simulink model "ffstudio_v2_6dof"  (R2026b)
settings: Solver=ode45  StopTime=25  MaxStep=0.02  RelTol=1e-6  AbsTol=1e-7
PostLoadFcn:
  | addpath(fileparts(fileparts(get_param('ffstudio_v2_6dof','FileName'))),'-begin');
model workspace (MAT data in the model file):
  ffStudioSimConfig.config.schemaVersion = 2
  ffStudioSimConfig.config.name = 'Blazhevski 6000 kg land-based firefighter'
  ffStudioSimConfig.config.designYear = 2036
  ffStudioSimConfig.config.payload_kg = 6000
  ffStudioSimConfig.config.crew_kg = 200
  ffStudioSimConfig.config.radius_km = 700
  ffStudioSimConfig.config.cruise_kmh = 580
  ffStudioSimConfig.config.cruiseAltitude_m = 5500
  ffStudioSimConfig.config.drop_kmh = 220
  ffStudioSimConfig.config.dropHeight_m = 40
  ffStudioSimConfig.config.pattern_min = 10
  ffStudioSimConfig.config.loiter_min = 45
  ffStudioSimConfig.config.loiter_kmh = 300
  ffStudioSimConfig.config.loiterAltitude_m = 1500
  ffStudioSimConfig.config.aspectRatio = 11.5
  ffStudioSimConfig.config.oswald = 0.8
  ffStudioSimConfig.config.wettedRatio = 5.5
  ffStudioSimConfig.config.KLD = 11
  ffStudioSimConfig.config.wingLoading_Nm2 = 3500
  ffStudioSimConfig.config.powerLoading_kWkg = 0.23
  ffStudioSimConfig.config.propEfficiency = 0.8
  ffStudioSimConfig.config.sfcCruise_kgkWh = 0.3
  ffStudioSimConfig.config.sfcLoiter_kgkWh = 0.36
  ffStudioSimConfig.config.takeoffFraction = 0.97
  ffStudioSimConfig.config.climbFraction = 0.985
  ffStudioSimConfig.config.descentFraction = 0.995
  ffStudioSimConfig.config.landingFraction = 0.995
  ffStudioSimConfig.config.reserveFactor = 1.06
  ffStudioSimConfig.config.emptyA = 1.442
  ffStudioSimConfig.config.emptyC = -0.0947
  ffStudioSimConfig.config.emptyScale = 1
  ffStudioSimConfig.config.sweepFactor = 1
  ffStudioSimConfig.config.gravity = 9.81
  ffStudioSimConfig.config.CLmaxClean = 1.6
  ffStudioSimConfig.config.CLmaxTakeoff = 2
  ffStudioSimConfig.config.CLmaxLanding = 2.4
  ffStudioSimConfig.config.deltaCDpattern = 0.06
  ffStudioSimConfig.config.deltaCDloiter = 0
  ffStudioSimConfig.config.powerLapseExponent = 0.7
  ffStudioSimConfig.config.engineCount = 2
  ffStudioSimConfig.config.takeoffTarget_m = 1000
  ffStudioSimConfig.config.landingTarget_m = 1000
  ffStudioSimConfig.config.climbTarget_ms = 8
  ffStudioSimConfig.config.oeiGradient = 0.024
  ffStudioSimConfig.config.muRoll = 0.03
  ffStudioSimConfig.config.muBrake = 0.35
  ffStudioSimConfig.config.deltaISA_K = 0
  ffStudioSimConfig.config.fieldAltitude_m = 0
  ffStudioSimConfig.config.taper = 0.45
  ffStudioSimConfig.config.tailArmH_m = 10.5
  ffStudioSimConfig.config.tailArmV_m = 10.2
  ffStudioSimConfig.config.VH = 1.106
  ffStudioSimConfig.config.VV = 0.0753
  ffStudioSimConfig.config.dihedral_deg = 2.75
  ffStudioSimConfig.config.aileronSpanFraction = 0.28
  ffStudioSimConfig.config.aileronChordFraction = 0.29
  ffStudioSimConfig.config.elevatorChordFraction = 0.34
  ffStudioSimConfig.config.rudderChordFraction = 0.335
  ffStudioSimConfig.config.cgEmpty_MAC = 0.28
  ffStudioSimConfig.config.cgCrew_MAC = -0.6
  ffStudioSimConfig.config.cgFuel_MAC = 0.3
  ffStudioSimConfig.config.cgWater_MAC = 0.3
  ffStudioSimConfig.config.cgMin_MAC = 0.15
  ffStudioSimConfig.config.cgMax_MAC = 0.4
  ffStudioSimConfig.config.dropDuration_s = 8
  ffStudioSimConfig.config.windNED_ms = [0 5 0]
  ffStudioSimConfig.config.parcelDiameter_m = 0.005
  ffStudioSimConfig.config.parcelCd = 0.47
  ffStudioSimConfig.config.waterDensity_kgm3 = 1000
  ffStudioSimConfig.config.releaseDown_ms = 0
  ffStudioSimConfig.config.releaseCount = 21
  ffStudioSimConfig.config.dyn.CL0 = 0.35
  ffStudioSimConfig.config.dyn.flapCL0 = 0.8
  ffStudioSimConfig.config.dyn.CLa = 5.2
  ffStudioSimConfig.config.dyn.CLde = 0.45
  ffStudioSimConfig.config.dyn.CLq = 3.5
  ffStudioSimConfig.config.dyn.Cm0 = 0
  ffStudioSimConfig.config.dyn.Cma = -0.8
  ffStudioSimConfig.config.dyn.Cmde = -1.1
  ffStudioSimConfig.config.dyn.Cmq = -12
  ffStudioSimConfig.config.dyn.CYb = -0.7
  ffStudioSimConfig.config.dyn.CYdr = 0.18
  ffStudioSimConfig.config.dyn.Clb = -0.1
  ffStudioSimConfig.config.dyn.Clp = -0.45
  ffStudioSimConfig.config.dyn.Clda = 0.18
  ffStudioSimConfig.config.dyn.Cnb = 0.15
  ffStudioSimConfig.config.dyn.Cnr = -0.2
  ffStudioSimConfig.config.dyn.Cndr = -0.12
  ffStudioSimConfig.config.dyn.radiusGyration_m = [5 6 7]
  ffStudioSimConfig.config.dyn.dropStart_s = 5
  ffStudioSimConfig.config.dyn.stopTime_s = 25
  ffStudioSimConfig.config.dyn.speedGain = 0.025
  ffStudioSimConfig.config.dyn.heightGain = 0.0015
  ffStudioSimConfig.config.dyn.pitchGain = 0.9
  ffStudioSimConfig.config.dyn.pitchRateGain = 0.5
  ffStudioSimConfig.config.dyn.rollGain = 0.6
  ffStudioSimConfig.config.dyn.rollRateGain = 0.3
  ffStudioSimConfig.config.dyn.yawRateGain = 0.4
  ffStudioSimConfig.config.dyn.fuelFlow_kgs = 0.2
  ffStudioSimConfig.config.dyn.autopilot = 1
  ffStudioSimConfig.config.dyn.engineOut = 0
  ffStudioSimConfig.config.dyn.elevatorPulse_deg = 0
  ffStudioSimConfig.config.dyn.pulseStart_s = 2
  ffStudioSimConfig.config.dyn.pulseDuration_s = 1
  ffStudioSimConfig.design.mtow_kg = 21965.2847244
  ffStudioSimConfig.design.fuel_kg = 3475.63176107
  ffStudioSimConfig.design.empty_kg = 12289.652954
  ffStudioSimConfig.design.payload_kg = 6000
  ffStudioSimConfig.design.crew_kg = 200
  ffStudioSimConfig.design.emptyFraction = 0.559503466867
  ffStudioSimConfig.design.payloadFraction = 0.273158307543
  ffStudioSimConfig.design.fuelFraction = 0.158232948249
  ffStudioSimConfig.design.wingArea_m2 = 61.5655551846
  ffStudioSimConfig.design.span_m = 26.6083423877
  ffStudioSimConfig.design.installedPower_kW = 5052.01548661
  ffStudioSimConfig.design.perEnginePower_kW = 2526.0077433
  ffStudioSimConfig.design.residual_kg = 9.29757698032e-06
  ffStudioSimConfig.design.mission.stations_kg = [21965.2847244; 21306.3261826; 20986.7312899; 20063.8378568; 19963.5186675; 19883.063741; 13883.063741; 13674.8177848; 13073.4664187; 13008.0990866; 12750.1375242; 12686.3868366]
  ffStudioSimConfig.design.mission.burn_kg = 3278.8978878
  ffStudioSimConfig.design.mission.fuel_kg = 3475.63176107
  ffStudioSimConfig.design.mission.extraReserve_kg = 196.733873268
  ffStudioSimConfig.design.mission.mode = 'report'
  ffStudioSimConfig.design.mission.table = table
  ffStudioSimConfig.design.mission.table.data{1} = [0; 1; 2; 3; 4; 5; 6; 7; 8; 9; 10]
  ffStudioSimConfig.design.mission.table.data{2} = [1; 2; 3; 4; 5; 6; 7; 8; 9; 10; 11]
  ffStudioSimConfig.design.mission.table.data{3} = ["Warm-up / taxi / take-off"; "Loaded climb"; "Outbound cruise"; "Descent to drop"; "Low-level pattern"; "Water release"; "Empty climb"; "Return cruise"; "Descent to reserve"; "Reserve loiter"; "Landing / taxi"]
  ffStudioSimConfig.design.mission.table.data{4} = [21965.2847244; 21306.3261826; 20986.7312899; 20063.8378568; 19963.5186675; 19883.063741; 13883.063741; 13674.8177848; 13073.4664187; 13008.0990866; 12750.1375242]
  ffStudioSimConfig.design.mission.table.data{5} = [21306.3261826; 20986.7312899; 20063.8378568; 19963.5186675; 19883.063741; 13883.063741; 13674.8177848; 13073.4664187; 13008.0990866; 12750.1375242; 12686.3868366]
  ffStudioSimConfig.design.mission.table.data{6} = [0.97; 0.985; 0.956024908294; 0.995; 0.995969902505; NaN; 0.985; 0.956024908294; 0.995; 0.980169157638; 0.995]
  ffStudioSimConfig.design.mission.table.data{7} = [658.958541731; 319.59489274; 922.89343308; 100.319189284; 80.4549265723; 0; 208.245956114; 601.35136615; 65.3673320935; 257.961562416; 63.7506876209]
  ffStudioSimConfig.design.mission.table.data{8} = [NaN; NaN; 4344.82758621; NaN; 600; 0; NaN; 4344.82758621; NaN; 2700; NaN]
  ffStudioSimConfig.design.mission.table.data{9} = [NaN; NaN; 3733.92048983; NaN; 1671.62217164; NaN; NaN; 3428.80965957; NaN; 932.367301197; NaN]
  ffStudioSimConfig.design.mission.table.data{10} = [NaN; NaN; 3404.69572299; NaN; 5038.44738929; NaN; NaN; 3404.69572299; NaN; 4559.620527; NaN]
  ffStudioSimConfig.design.mission.table.data{11} = [NaN; NaN; 15.9059737206; NaN; 11.1341816044; NaN; NaN; 15.9059737206; NaN; 13.774573242; NaN]
  ffStudioSimConfig.design.mission.table.data{12} = [NaN; NaN; 0.369620967159; NaN; 1.39601581167; NaN; NaN; 0.240842621252; NaN; 0.564188541196; NaN]
  ffStudioSimConfig.design.mission.table.ndims = 2
  ffStudioSimConfig.design.mission.table.nrows = 11
  ffStudioSimConfig.design.mission.table.nvars = 12
  ffStudioSimConfig.design.mission.table.varnames = {'From', 'To', 'Phase', 'Start_kg', 'End_kg', 'MassFraction', 'FuelBurn_kg', 'Duration_s', 'RequiredPower_kW', 'AvailablePower_kW', 'LD', 'CL'}
  ffStudioSimConfig.design.mission.table.props.CustomProps = struct()
  ffStudioSimConfig.design.mission.table.props.VariableCustomProps = struct()
  ffStudioSimConfig.design.mission.table.props.versionSavedFrom = 5
  ffStudioSimConfig.design.mission.table.props.minCompatibleVersion = 1
  ffStudioSimConfig.design.mission.table.props.incompatibilityMsg = ''
  ffStudioSimConfig.design.mission.table.props.VersionSavedFrom = 5
  ffStudioSimConfig.design.mission.table.props.useVariableNamesOriginal = 0
  ffStudioSimConfig.design.mission.table.props.useVariableNames2048 = 0
  ffStudioSimConfig.design.mission.table.props.useDimensionNamesOriginal = 0
  ffStudioSimConfig.design.mission.table.props.useDimensionNames2048 = 0
  ffStudioSimConfig.design.mission.table.props.Description = ''
  ffStudioSimConfig.design.mission.table.props.VariableNamesOriginal = {}
  ffStudioSimConfig.design.mission.table.props.VariableNames2048 = {}
  ffStudioSimConfig.design.mission.table.props.DimensionNames = {'Row', 'Variables'}
  ffStudioSimConfig.design.mission.table.props.DimensionNamesOriginal = {}
  ffStudioSimConfig.design.mission.table.props.DimensionNames2048 = {}
  ffStudioSimConfig.design.mission.table.props.UserData = []
  ffStudioSimConfig.design.mission.table.props.VariableDescriptions = {}
  ffStudioSimConfig.design.mission.table.props.VariableUnits = {}
  ffStudioSimConfig.design.mission.table.props.VariableContinuity = {}
  ffStudioSimConfig.design.mission.note = 'Climb/ground/descent/landing retain empirical report fractions. Requested speeds are checked against power availability, not automatically reduced.'
  ffStudioSimConfig.design.mode = 'report'
  ffStudioSimConfig.design.iteration = table
  ffStudioSimConfig.design.iteration.data = {[7200; 10128.8135593; 13057.6271186; 15986.440678; 18915.2542373; 21844.0677966; 24772.8813559; 27701.6949153; 30630.5084746; 33559.3220339; 36488.1355932; 39416.9491525; 42345.7627119; 45274.5762712; 48203.3898305; 51132.2033898; 54061.0169492; 56989.8305085; 59918.6440678; 62847.4576271; 65776.2711864; 68705.0847458; 71633.8983051; 74562.7118644; 77491.5254237; 80420.3389831; 83349.1525424; 86277.9661017; 89206.779661; 92135.5932203; 95064.4067797; 97993.220339; 100922.033898; 103850.847458; 106779.661017; 109708.474576; 112637.288136; 115566.101695; 118494.915254; 121423.728814; 124352.542373; 127281.355932; 130210.169492; 133138.983051; 136067.79661; 138996.610169; 141925.423729; 144854.237288; 147783.050847; 150711.864407; 153640.677966; 156569.491525; 159498.305085; 162427.118644; 165355.932203; 168284.745763; 171213.559322; 174142.372881; 177071.186441; 180000], [-4247.98280058; -3476.62310134; -2660.82656192; -1811.60280364; -935.682153221; -37.5963688103; 879.400809852; 1812.86331818; 2760.88747666; 3721.95108369; 4694.81021348; 5678.43002022; 6671.93663348; 7674.58269474; 8685.72203078; 9704.79063173; 10731.2920919; 11764.7862807; 12804.8803977; 13851.2218175; 14903.4922995; 15961.4032536; 17024.691831; 18093.1176703; 19166.4601655; 20244.5161577; 21327.09797; 22414.0317252; 23505.1558976; 24600.3200588; 25699.383787; 26802.2157136; 27908.6926868; 29018.6990337; 30132.1259087; 31248.870714; 32368.8365841; 33491.9319245; 34618.0699992; 35747.1685587; 36879.1495058; 38013.9385932; 39151.4651492; 40291.6618292; 41434.4643893; 42579.8114801; 43727.6444577; 44877.9072114; 46030.5460052; 47185.509332; 48342.7477802; 49502.2139094; 50663.8621371; 51827.6486328; 52993.5312202; 54161.469287; 55331.4237003; 56503.3567285; 57677.2319685; 58853.0142775]}
  ffStudioSimConfig.design.iteration.ndims = 2
  ffStudioSimConfig.design.iteration.nrows = 60
  ffStudioSimConfig.design.iteration.nvars = 2
  ffStudioSimConfig.design.iteration.varnames = {'AssumedMTOW_kg', 'ClosureResidual_kg'}
  ffStudioSimConfig.design.iteration.props.CustomProps = struct()
  ffStudioSimConfig.design.iteration.props.VariableCustomProps = struct()
  ffStudioSimConfig.design.iteration.props.versionSavedFrom = 5
  ffStudioSimConfig.design.iteration.props.minCompatibleVersion = 1
  ffStudioSimConfig.design.iteration.props.incompatibilityMsg = ''
  ffStudioSimConfig.design.iteration.props.VersionSavedFrom = 5
  ffStudioSimConfig.design.iteration.props.useVariableNamesOriginal = 0
  ffStudioSimConfig.design.iteration.props.useVariableNames2048 = 0
  ffStudioSimConfig.design.iteration.props.useDimensionNamesOriginal = 0
  ffStudioSimConfig.design.iteration.props.useDimensionNames2048 = 0
  ffStudioSimConfig.design.iteration.props.Description = ''
  ffStudioSimConfig.design.iteration.props.VariableNamesOriginal = {}
  ffStudioSimConfig.design.iteration.props.VariableNames2048 = {}
  ffStudioSimConfig.design.iteration.props.DimensionNames = {'Row', 'Variables'}
  ffStudioSimConfig.design.iteration.props.DimensionNamesOriginal = {}
  ffStudioSimConfig.design.iteration.props.DimensionNames2048 = {}
  ffStudioSimConfig.design.iteration.props.UserData = []
  ffStudioSimConfig.design.iteration.props.VariableDescriptions = {}
  ffStudioSimConfig.design.iteration.props.VariableUnits = {}
  ffStudioSimConfig.design.iteration.props.VariableContinuity = {}
  ffStudioSimConfig.polar.LDmax = 15.9059737206
  ffStudioSimConfig.polar.k = 0.0345989006722
  ffStudioSimConfig.polar.CD0 = 0.0285599332145
  ffStudioSimConfig.polar.CLbest = 0.908547094342
  ffStudioSimConfig.polar.CL = [0; 0.01; 0.02; 0.03; 0.04; 0.05; 0.06; 0.07; 0.08; 0.09; 0.1; 0.11; 0.12; 0.13; 0.14; 0.15; 0.16; 0.17; 0.18; 0.19; 0.2; 0.21; 0.22; 0.23; 0.24; 0.25; 0.26; 0.27; 0.28; 0.29; 0.3; 0.31; 0.32; 0.33; 0.34; 0.35; 0.36; 0.37; 0.38; 0.39; 0.4; 0.41; 0.42; 0.43; 0.44; 0.45; 0.46; 0.47; 0.48; 0.49; 0.5; 0.51; 0.52; 0.53; 0.54; 0.55; 0.56; 0.57; 0.58; 0.59; 0.6; 0.61; 0.62; 0.63; 0.64; 0.65; 0.66; 0.67; 0.68; 0.69; 0.7; 0.71; 0.72; 0.73; 0.74; 0.75; 0.76; 0.77; 0.78; 0.79; 0.8; 0.81; 0.82; 0.83; 0.84; 0.85; 0.86; 0.87; 0.88; 0.89; 0.9; 0.91; 0.92; 0.93; 0.94; 0.95; 0.96; 0.97; 0.98; 0.99; 1; 1.01; 1.02; 1.03; 1.04; 1.05; 1.06; 1.07; 1.08; 1.09; 1.1; 1.11; 1.12; 1.13; 1.14; 1.15; 1.16; 1.17; 1.18; 1.19; 1.2; 1.21; 1.22; 1.23; 1.24; 1.25; 1.26; 1.27; 1.28; 1.29; 1.3; 1.31; 1.32; 1.33; 1.34; 1.35; 1.36; 1.37; 1.38; 1.39; 1.4; 1.41; 1.42; 1.43; 1.44; 1.45; 1.46; 1.47; 1.48; 1.49; 1.5; 1.51; 1.52; 1.53; 1.54; 1.55; 1.56; 1.57; 1.58; 1.59; 1.6; 1.61; 1.62; 1.63; 1.64; 1.65; 1.66; 1.67; 1.68; 1.69; 1.7; 1.71; 1.72; 1.73; 1.74; 1.75; 1.76; 1.77; 1.78; 1.79; 1.8; 1.81; 1.82; 1.83; 1.84; 1.85; 1.86; 1.87; 1.88; 1.89; 1.9; 1.91; 1.92; 1.93; 1.94; 1.95; 1.96; 1.97; 1.98; 1.99; 2; 2.01; 2.02; 2.03; 2.04; 2.05; 2.06; 2.07; 2.08; 2.09; 2.1; 2.11; 2.12; 2.13; 2.14; 2.15; 2.16; 2.17; 2.18; 2.19; 2.2; 2.21; 2.22; 2.23; 2.24; 2.25; 2.26; 2.27; 2.28; 2.29; 2.3; 2.31; 2.32; 2.33; 2.34; 2.35; 2.36; 2.37; 2.38; 2.39; 2.4; 2.41; 2.42; 2.43; 2.44; 2.45; 2.46; 2.47; 2.48; 2.49; 2.5]
  ffStudioSimConfig.polar.CD = [0.0285599332145 0.0285633931045 0.0285737727747 0.0285910722251 0.0286152914555 0.0286464304661 0.0286844892569 0.0287294678277 0.0287813661788 0.0288401843099 0.0289059222212 0.0289785799126 ... (251 elements, 251x1)]
  ffStudioSimConfig.polar.LD = [0 0.350098462161 0.699942571731 1.04927859172 1.3978540132 1.74541816158 2.09172279355 2.43652268186 2.77957618492 3.12064579869 3.45949868801 3.79590719531 ... (251 elements, 251x1)]
  ffStudioSimConfig.geometry.wingArea_m2 = 61.5655551846
  ffStudioSimConfig.geometry.span_m = 26.6083423877
  ffStudioSimConfig.geometry.rootChord_m = 3.19140538384
  ffStudioSimConfig.geometry.tipChord_m = 1.43613242273
  ffStudioSimConfig.geometry.MAC_m = 2.42473443531
  ffStudioSimConfig.geometry.MACspanStation_m = 5.81101730307
  ffStudioSimConfig.geometry.horizontalTail_m2 = 15.7241728175
  ffStudioSimConfig.geometry.verticalTail_m2 = 12.0934558907
  ffStudioSimConfig.geometry.aileronSpanEach_m = 3.72516793428
  ffStudioSimConfig.geometry.aileronChordAtMAC_m = 0.703172986239
  ffStudioSimConfig.geometry.elevatorChordFraction = 0.34
  ffStudioSimConfig.geometry.rudderChordFraction = 0.335
  ffStudioSimConfig.geometry.dihedral_deg = 2.75
  ffStudioSimConfig.geometry.tankVolume_m3 = 6
  ffStudioSimConfig.geometry.note = 'Tail/control geometry is preliminary. No measured neutral point, downwash or stability derivatives supplied.'
  ffStudioSimConfig.initialMass_kg = 19883.063741
  ffStudioSimConfig.targetSpeed_ms = 61.1111111111
  ffStudioSimConfig.targetHeight_m = 40
  ffStudioSimConfig.trimAlpha_rad = 0.0478141957587
  ffStudioSimConfig.trimElevator_rad = -0.0347739605518
  ffStudioSimConfig.trimThrottle = 0.329485099126
  ffStudioSimConfig.initialEuler_rad = [0 0.0478141957587 0]
  ffStudioSimConfig.initialVelocityBody_ms = [61.0412683897 5 2.92086538701]
  ffStudioSimConfig.initialPositionNED_m = [0 0 -40]
  ffStudioSimConfig.initialRates_rads = [0 0 0]
libraries: simulink x1
settings Model: Creator=blaze  LastModifiedBy=blaze

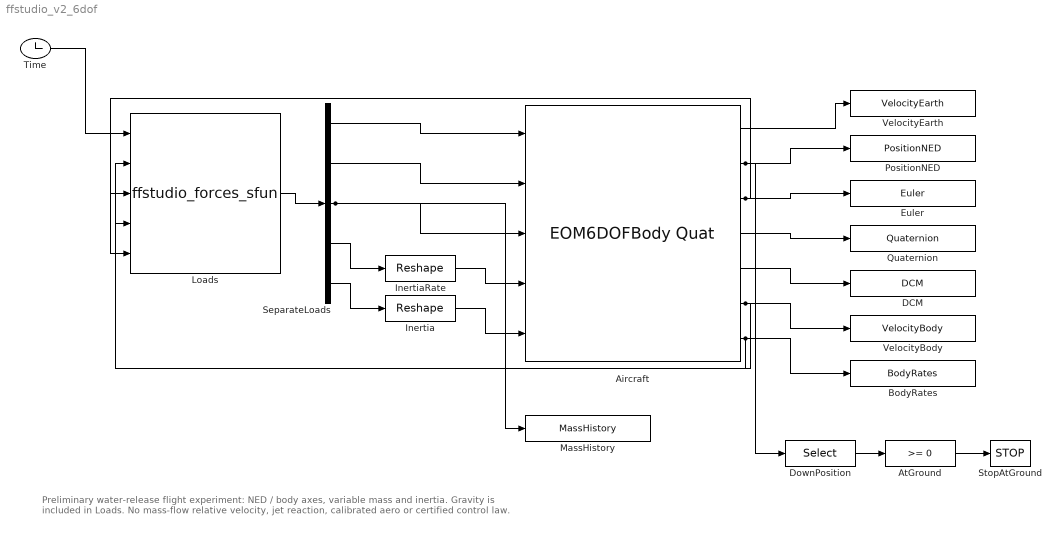
== system ffstudio_v2_6dof ==
  note: Preliminary water-release flight experiment: NED / body axes, variable mass and inertia.
      | Gravity is included in Loads. No mass-flow relative velocity, jet reaction, calibrated aero or certified control law.
  Aircraft : EOM6DOFBodyQuat  mtype=Custom Variable  xme_0=[0 0 -40]  Vm_0=[61.0412683897176 5 2.920865387009504]  eul_0=[0 0.04781419575868457 0]
  AtGround : simulink/Logic and Bit Operations/Compare To Constant  relop=>=  const=0  OutDataTypeStr=boolean
  BodyRates : ToWorkspace  VariableName=BodyRates  SaveFormat=Timeseries  SampleTime=-1
  DCM : ToWorkspace  VariableName=DCM  SaveFormat=Timeseries  SampleTime=-1
  DownPosition : Selector  InputPortWidth=3  IndexOptions=Index vector (dialog)  Indices=3  OutputSizes=1
  Euler : ToWorkspace  VariableName=Euler  SaveFormat=Timeseries  SampleTime=-1
  Inertia : Reshape  OutputDimensionality=Customize  OutputDimensions=[3 3]
  InertiaRate : Reshape  OutputDimensionality=Customize  OutputDimensions=[3 3]
  Loads : M-S-Function  FunctionName=ffstudio_forces_sfun  Parameters=ffStudioSimConfig
  MassHistory : ToWorkspace  VariableName=MassHistory  SaveFormat=Timeseries  SampleTime=-1
  PositionNED : ToWorkspace  VariableName=PositionNED  SaveFormat=Timeseries  SampleTime=-1
  Quaternion : ToWorkspace  VariableName=Quaternion  SaveFormat=Timeseries  SampleTime=-1
  SeparateLoads : Demux  Outputs=[3 3 1 9 9]
  StopAtGround : Stop
  Time : Clock
  VelocityBody : ToWorkspace  VariableName=VelocityBody  SaveFormat=Timeseries  SampleTime=-1
  VelocityEarth : ToWorkspace  VariableName=VelocityEarth  SaveFormat=Timeseries  SampleTime=-1
  wires:
  Time/1 -> Loads/1
  Loads/1 -> SeparateLoads/1
  SeparateLoads/1 -> Aircraft/1
  SeparateLoads/2 -> Aircraft/2
  SeparateLoads/3 -> Aircraft/3, MassHistory/1
  SeparateLoads/4 -> InertiaRate/1
  InertiaRate/1 -> Aircraft/4
  SeparateLoads/5 -> Inertia/1
  Inertia/1 -> Aircraft/5
  Aircraft/6 -> Loads/2, VelocityBody/1
  Aircraft/3 -> Loads/3, Euler/1
  Aircraft/7 -> Loads/4, BodyRates/1
  Aircraft/2 -> Loads/5, PositionNED/1, DownPosition/1
  Aircraft/1 -> VelocityEarth/1
  Aircraft/4 -> Quaternion/1
  Aircraft/5 -> DCM/1
  DownPosition/1 -> AtGround/1
  AtGround/1 -> StopAtGround/1
